simulink model "extra_tip_sim"  (Simulink 9.0)
settings: Solver=FixedStepDiscrete  StartTime=start_time  StopTime=stop_time  FixedStep=0.020  RelTol=1e-3  EnableMultiTasking=on
InitFcn:
  | extra_tip_sim_init
values from neighbouring files (symbols this model uses):
  bucketAngle = WeighDebug_TOAbucket_angle_t27    [extra_tip_sim_init.m]
  imuX = WeighDebug_TOAeef_imu_accelX_t27    [extra_tip_sim_init.m]    (also in imu_pitch_cal_sim_init.m = WeighDebug_TOAeef_imu_accelX_t194)
  imuY = WeighDebug_TOAeef_imu_accelY_t27    [extra_tip_sim_init.m]    (also in imu_pitch_cal_sim_init.m = WeighDebug_TOAeef_imu_accelY_t194)
  imuZ = WeighDebug_TOAeef_imu_accelZ_t27    [extra_tip_sim_init.m]    (also in imu_pitch_cal_sim_init.m = WeighDebug_TOAeef_imu_accelZ_t194)
  liftAngle = WeighDebug_TOAlift_angle_t27    [extra_tip_sim_init.m]    (also in imu_pitch_cal_sim_init.m = WeighDebug_TOAlift_angle_t194)
  liftCmd = WeighDebug_TOAlift_valve_cmd_t27    [extra_tip_sim_init.m]
  liftCylLength = WeighDebug_LiftCylNormLen_t27    [extra_tip_sim_init.m]    (also in imu_pitch_cal_sim_init.m = WeighDebug_LiftCylLenghtNorm_Val_t194)
  liftCylPress = WeighDebug_LiftCylPres_t27    [extra_tip_sim_init.m]    (also in imu_pitch_cal_sim_init.m = WeighDebug_LiftCylPres_t194)
  payloadTarget = TOAtestPts_toa_payload_target_final_t27    [extra_tip_sim_init.m]
  steerAng = WeighDebug_TOAsteering_angle_t27    [extra_tip_sim_init.m]    (also in imu_pitch_cal_sim_init.m = WeighDebug_TOAsteering_angle_t194)
  tiltCmd = WeighDebug_TOAtilt_valve_cmd_t27    [extra_tip_sim_init.m]
  tiltExt = WeighDebug_TOAtilt_extension_t27    [extra_tip_sim_init.m]    (also in imu_pitch_cal_sim_init.m = WeighDebug_TOAtilt_extension_t194)
  tiltHePress = WeighDebug_TOAtilt_he_pressure_t27    [extra_tip_sim_init.m]    (also in imu_pitch_cal_sim_init.m = WeighDebug_TOAtilt_he_pressure_t194)
  tiltRePress = WeighDebug_TOAtilt_re_pressure_t27    [extra_tip_sim_init.m]    (also in imu_pitch_cal_sim_init.m = WeighDebug_TOAtilt_re_pressure_t194)
  time = t27    [extra_tip_sim_init.m]    (also in imu_pitch_cal_sim_init.m = t194)
  time2 = t27    [extra_tip_sim_init.m]    (also in imu_pitch_cal_sim_init.m = t194)
  time3 = t28    [extra_tip_sim_init.m]
  toolMass = WeighDebug_TOAtool_mass_t28    [extra_tip_sim_init.m]
  unlatchTrigger = WeighDebug_TOAunlatch_trigger_t27    [extra_tip_sim_init.m]
undefined symbols (not defined in the file or in its folder): g, timestep, TipAssistLiveWeighStatus_t, TipAssistPfwStatus_t, toa_appNumber, toa_imu_lpf_cutoff_hz, toa_imuBasicOrient, toa_liftBoreDia, toa_liveLpfCutoffHz, toa_pfwLpfCutoffHz, toa_ratedPayload, toa_tiltBoreDia, toa_tiltNumCyl, toa_tiltRodDia, toa_toolBcLength
libraries: simulink x28, lib_CATutils_Utilities_ApplyName_v2 x15, lib_CATutils_Filters_1Pole_LowPass x3, tip_assist_lib x3, lib_CATutils_Timer_Countdown x3, simulink_extras x2, lib_CATutils_Override x1
(part 2 of 3)

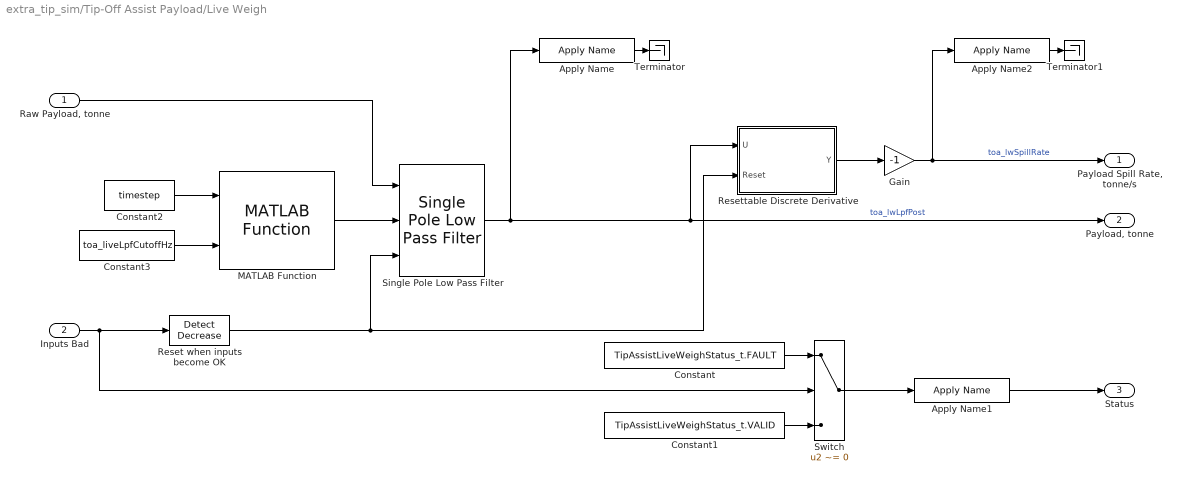
== system extra_tip_sim/Tip-Off Assist Payload/Live Weigh ==
  "Raw Payload, tonne" : Inport
  Inputs Bad : Inport  Port=2
  Apply Name : lib_CATutils_Utilities_ApplyName_v2/Apply Name  sigLabel='toa_lwLpfPost2'  enTst=true
  Apply Name1 : lib_CATutils_Utilities_ApplyName_v2/Apply Name  sigLabel='toa_lwStatus'  enTst=true
  Apply Name2 : lib_CATutils_Utilities_ApplyName_v2/Apply Name  sigLabel='toa_lwSpillRate2'  enTst=true
  Constant : Constant  Value=TipAssistLiveWeighStatus_t.FAULT  SampleTime=-1
  Constant1 : Constant  Value=TipAssistLiveWeighStatus_t.VALID  SampleTime=-1
  Constant2 : Constant  Value=timestep  SampleTime=timestep
  Constant3 : Constant  Value=toa_liveLpfCutoffHz  SampleTime=timestep
  Gain : Gain  Gain=-1
  MATLAB Function : tip_assist_lib/MATLAB Function
      settings: SourceProductName=Stateflow  SourceProductBaseCode=SF
  Reset when inputs become OK : simulink/Logic and Bit Operations/Detect Decrease  vinit=0  OutDataTypeStr=boolean
  Resettable Discrete Derivative : Subsystem  mask(Discrete Derivative){gainval=1, InputProcessing=Inherited, OutMin=[], OutMax=[], OutDataTypeStr=single, OutputDataTypeScalingMode=single, OutDataType=fixdt(1, 16), OutScaling=2^-10, LockScale=off, RndMeth=Floor, DoSatur=off}
      mask prompts: gainval "Simulink:masks:GainValue_MP"; InputProcessing "Simulink:masks:InputProcessing_MP"; OutMin "Simulink:masks:OutputMinimum_MP"; OutMax "Simulink:masks:OutputMaximum_MP"; OutDataTypeStr "Simulink:masks:OutputDataType_MP"; OutputDataTypeScalingMode "Simulink:masks:OutputDataTypeMode_MP"; OutDataType "Simulink:masks:OutputDataTypeegFixdt116Fixdtsingle_MP"; OutScaling "Simulink:masks:OutputScalingSlopeEg29OrSlopeBias_MP"; LockScale "Simulink:masks:LockOutputDataTypeAgainstFxpTools_MP"; RndMeth "Simulink:masks:IntegerRoundingMode_MP"; DoSatur "Simulink:masks:SaturateToMaxOrMinWhenOverflowsOccur_MP"
      mask help: Simulink:masks:DiscreteDerivative_MD
      mask init:
      | blkH = gcbh;
      | blkName = getfullname(blkH);
      | 
      | if (gainval == 0.0)
      |     %avoid divide by zero warning
      |     inverseGainval = inf;
      | else
      |     inverseGainval = 1.0/double(gainval);
      | end
      | 
      | if isequal(OutDataTypeStr, 'Inherit: Inherit via internal rule')
      |     diffDT   = 'Inherit: Inherit via back propagation';
      |     tsampDT  = 'Inherit: Inherit via internal rule';
      |     tsampImp = 'Offline Scaling Adjustment';
      | else    
      |     diffDT   = OutDataTypeStr;
      |     tsampDT  = 'Inherit: Inherit via back propagation';
      |     tsampImp = 'Online Calculations';
      | end
      | 
      | if ~strcmp(get_param(bdroot(blkH),'SimulationStatus'), 'running')
      |     set_param([blkName,'/Diff'], ...
      |               'RndMeth',RndMeth, ...
      | 	          'DoSatur',DoSatur);
      |     set_param([blkName,'/TSamp'], ...
      |               'OutDataTypeStr',tsampDT, ...
      |               'RndMeth',RndMeth, ...
      |               'DoSatur',DoSatur, ...
      |               'TsampMathImp',tsampImp);
      | end
      | 
      | set_param([blkName,'/Resettable Delay'], ...
      | 	'InputProcessing',InputProcessing);
      mask TypeOptions InputProcessing: Simulink:masks:ColumnsAsChannelsFrameBased | Simulink:masks:ElementsAsChannelsSampleBased | Simulink:masks:Inherited
      mask Callback OutDataTypeStr: fixptdialog(gcbh)
      mask TypeOptions OutputDataTypeScalingMode: double | single | int8 | uint8 | int16 | uint16 | int32 | uint32 | Specify via dialog | Inherit via internal rule | Inherit via back propagation
      mask Callback OutputDataTypeScalingMode: fixptdialog(gcbh)
      mask Callback OutDataType: fixptdialog(gcbh)
      mask TypeOptions RndMeth: Simulink:masks:Ceiling | Simulink:masks:Convergent | Simulink:masks:Floor | Simulink:masks:Nearest | Simulink:masks:Round | Simulink:masks:Simplest | Simulink:masks:Zero
      mask Display: text(0.5, 0.5, 'K (z-1)', 'horizontalAlignment', 'center', 'verticalAlignment', 'bottom');text(0.5, 0.5, 'Ts z', 'horizontalAlignment', 'center', 'verticalAlignment', 'top');plot([0.3 0.7],[0.5 0.5]);
  Single Pole Low Pass Filter : lib_CATutils_Filters_1Pole_LowPass/Single Pole Low Pass Filter  extFactor=on  extReset=on  incIntWordSize=off  mainInternalRes=off  filtFactor=.0001
  Switch : Switch  Criteria=u2 ~= 0
  Terminator : Terminator
  Terminator1 : Terminator
  "Payload Spill Rate, tonne/s" : Outport
  "Payload, tonne" : Outport  Port=2
  Status : Outport  Port=3
  wires:
  Apply Name2/1 -> Terminator1/1
  Apply Name/1 -> Terminator/1
  Gain/1 -> Apply Name2/1, "Payload Spill Rate, tonne/s"/1  "toa_lwSpillRate"
  Resettable Discrete Derivative/1(Y) -> Gain/1
  Apply Name1/1 -> Status/1
  Constant3/1 -> MATLAB Function/2
  Constant2/1 -> MATLAB Function/1
  Switch/1 -> Apply Name1/1
  Constant1/1 -> Switch/3
  Constant/1 -> Switch/1
  "Raw Payload, tonne"/1 -> Single Pole Low Pass Filter/1
  Inputs Bad/1 -> Reset when inputs become OK/1, Switch/2
  Reset when inputs become OK/1 -> Single Pole Low Pass Filter/3, Resettable Discrete Derivative/2(Reset)
  MATLAB Function/1 -> Single Pole Low Pass Filter/2
  Single Pole Low Pass Filter/1 -> "Payload, tonne"/1, Resettable Discrete Derivative/1(U), Apply Name/1  "toa_lwLpfPost"

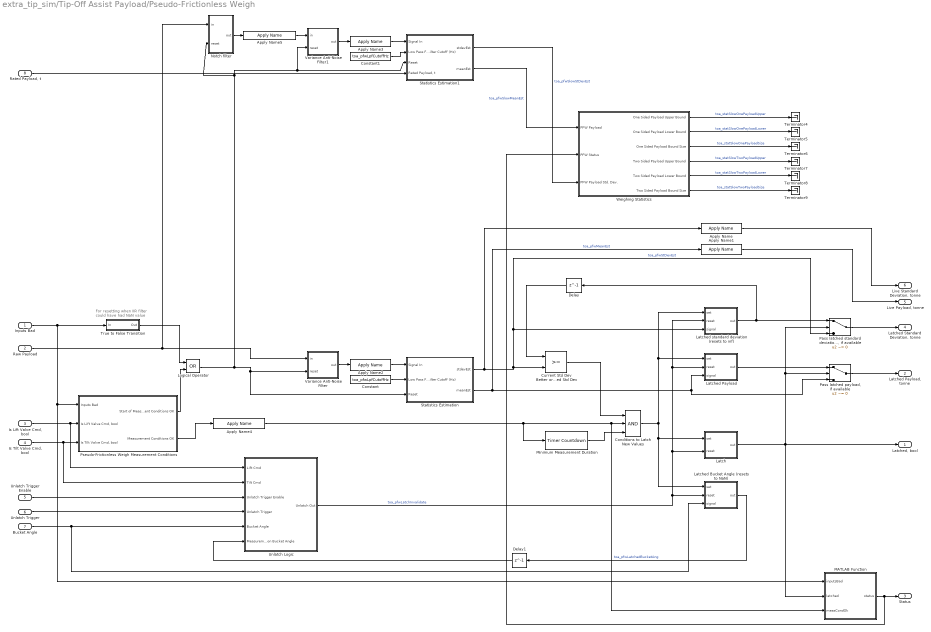
== system extra_tip_sim/Tip-Off Assist Payload/Pseudo-Frictionless Weigh ==
  note: For resetting when IIR filter could have had NaN value
  Inputs Bad : Inport
  Raw Payload : Inport  Port=2
  "Is Lift Valve Cmd, bool" : Inport  Port=3
  "Is Tilt Valve Cmd, bool" : Inport  Port=4
  Unlatch Trigger Enable : Inport  Port=5
  Unlatch Trigger : Inport  Port=6
  Bucket Angle : Inport  Port=7
  "Rated Payload, t" : Inport  Port=8
  Apply Name : lib_CATutils_Utilities_ApplyName_v2/Apply Name  sigLabel='toa_pfwLiveStDev'  enTst=true
  Apply Name1 : lib_CATutils_Utilities_ApplyName_v2/Apply Name  sigLabel='toa_pfwLiveMean'  enTst=true
  Apply Name2 : lib_CATutils_Utilities_ApplyName_v2/Apply Name  sigLabel='toa_pfwPayloadFilt'  enTst=true
  Apply Name3 : lib_CATutils_Utilities_ApplyName_v2/Apply Name  sigLabel='toa_pfwPayloadFilt'  enTst=true
  Apply Name4 : lib_CATutils_Utilities_ApplyName_v2/Apply Name  sigLabel='toa_pfwConditionsOk'  enTst=true
  Apply Name5 : lib_CATutils_Utilities_ApplyName_v2/Apply Name  sigLabel='toa_pfwPayloadNotchPost'  enTst=true
  Conditions to Latch New Values : Logic  Inputs=3
  Constant : Constant  Value=toa_pfwLpfCutoffHz
  Constant1 : Constant  Value=toa_pfwLpfCutoffHz
  Current Std Dev Better or Equal to Previously Latched Std Dev : RelationalOperator  RndMeth=Nearest  InputSameDT=on
  Delay : Delay  DelayLength=1
  Delay1 : Delay  DelayLength=1
  Latch : Subsystem  mask{mskInitialOut=0}
      mask prompts: mskInitialOut "Initial Output"
  Latched Bucket Angle (resets to NaN) : Subsystem  mask{mskInitialOut=single(nan)}
      mask prompts: mskInitialOut "Initial Output and Reset Value"
  Latched Payload : Subsystem  mask{mskInitialOut=nan}
      mask prompts: mskInitialOut "Initial Output and Reset Value"
  Latched standard deviation (resets to inf) : Subsystem  mask{mskInitialOut=single(inf)}
      mask prompts: mskInitialOut "Initial Output and Reset Value"
  Logical Operator : Logic  Operator=OR  AllPortsSameDT=off  OutDataTypeStr=boolean
  MATLAB Function : MATLAB Function  TreatAsAtomicUnit=on
  Minimum Measurement Duration : lib_CATutils_Timer_Countdown/Timer Countdown  initTime=toa_pfw_min_meas_duration  maxTime=400  timingInput=True  expiredOutput=True  initState=False
  Notch filter : Subsystem
  "Pass latched payload, if available" : Switch  Criteria=u2 ~= 0
  "Pass latched standard deviation, if available" : Switch  Criteria=u2 ~= 0
  Pseudo-Frictionless Weigh Measurement Conditions : Subsystem
  Statistics Estimation : Subsystem
  Statistics Estimation1 : Subsystem
  Terminator{4..9} (6 alike) : Terminator
  True to False Transition : Subsystem
  Unlatch Logic : Subsystem
  Variance Anti-Noise Filter : Subsystem
  Variance Anti-Noise Filter1 : Subsystem
  Weighing Statistics : Subsystem
  "Latched, bool" : Outport
  "Latched Payload, tonne" : Outport  Port=2
  Status : Outport  Port=3
  "Latched Standard Deviation, tonne" : Outport  Port=4
  "Live Payload, tonne" : Outport  Port=5
  "Live Standard Deviation, tonne" : Outport  Port=6
  wires:
  Apply Name1/1 -> "Live Payload, tonne"/1
  Apply Name/1 -> "Live Standard Deviation, tonne"/1
  Unlatch Trigger Enable/1 -> Unlatch Logic/3(Unlatch Trigger Enable)
  Delay1/1 -> Unlatch Logic/6(Measurement Condition Bucket Angle)
  Unlatch Trigger/1 -> Unlatch Logic/4(Unlatch Trigger)
  Latched Bucket Angle (resets to NaN)/1(out) -> Delay1/1  "toa_pfwLatchedBucketAng"
  Bucket Angle/1 -> Unlatch Logic/5(Bucket Angle), Latched Bucket Angle (resets to NaN)/3(signal)
  Logical Operator/1 -> Notch filter/2(reset), Variance Anti-Noise Filter1/2(reset), Statistics Estimation1/3(Reset), Statistics Estimation/3(Reset), Variance Anti-Noise Filter/2(reset)
  True to False Transition/1(Out) -> Logical Operator/1
  Constant/1 -> Statistics Estimation/2(Low Pass Filter Cutoff (Hz))
  Inputs Bad/1 -> True to False Transition/1(In), Pseudo-Frictionless Weigh Measurement Conditions/1(Inputs Bad), MATLAB Function/1(inputsBad)
  "Is Lift Valve Cmd, bool"/1 -> Pseudo-Frictionless Weigh Measurement Conditions/2("Is Lift Valve Cmd, bool"), Unlatch Logic/1(Lift Cmd)
  Conditions to Latch New Values/1 -> Latched standard deviation (resets to inf)/1(set), Latched Payload/1(set), Latch/1(set), Latched Bucket Angle (resets to NaN)/1(set)
  Latch/1(out) -> MATLAB Function/2(latched), "Latched, bool"/1, "Pass latched payload, if available"/2, "Pass latched standard deviation, if available"/2
  Latched Payload/1(out) -> "Pass latched payload, if available"/1
  Latched standard deviation (resets to inf)/1(out) -> "Pass latched standard deviation, if available"/1, Delay/1
  Minimum Measurement Duration/1 -> Conditions to Latch New Values/3
  Current Std Dev Better or Equal to Previously Latched Std Dev/1 -> Conditions to Latch New Values/1
  Delay/1 -> Current Std Dev Better or Equal to Previously Latched Std Dev/1
  Pseudo-Frictionless Weigh Measurement Conditions/2(Measurement Conditions OK) -> Apply Name4/1
  Pseudo-Frictionless Weigh Measurement Conditions/1(Start of Measurement Conditions OK) -> Logical Operator/2
  "Is Tilt Valve Cmd, bool"/1 -> Pseudo-Frictionless Weigh Measurement Conditions/3("Is Tilt Valve Cmd, bool"), Unlatch Logic/2(Tilt Cmd)
  Variance Anti-Noise Filter/1(out) -> Apply Name2/1
  "Pass latched payload, if available"/1 -> "Latched Payload, tonne"/1
  "Pass latched standard deviation, if available"/1 -> "Latched Standard Deviation, tonne"/1
  MATLAB Function/1(status) -> Weighing Statistics/2(PFW Status), Status/1
  Statistics Estimation/1(stdevEst) -> Current Std Dev Better or Equal to Previously Latched Std Dev/2, Latched standard deviation (resets to inf)/3(signal), "Pass latched standard deviation, if available"/3, Apply Name/1  "toa_pfwStDevEst"
  Statistics Estimation/2(meanEst) -> "Pass latched payload, if available"/3, Latched Payload/3(signal), Apply Name1/1  "toa_pfwMeanEst"
  Apply Name2/1 -> Statistics Estimation/1(Signal In)
  Raw Payload/1 -> Notch filter/1(in), Variance Anti-Noise Filter/1(in)
  Apply Name4/1 -> Minimum Measurement Duration/1, MATLAB Function/3(measCondOk), Conditions to Latch New Values/2
  Unlatch Logic/1(Unlatch Out) -> Latched Bucket Angle (resets to NaN)/2(reset), Latch/2(reset), Latched Payload/2(reset), Latched standard deviation (resets to inf)/2(reset)  "toa_pfwLatchInvalidate"
  Apply Name5/1 -> Variance Anti-Noise Filter1/1(in)
  Notch filter/1(out) -> Apply Name5/1
  Variance Anti-Noise Filter1/1(out) -> Apply Name3/1
  Constant1/1 -> Statistics Estimation1/2(Low Pass Filter Cutoff (Hz))
  Apply Name3/1 -> Statistics Estimation1/1(Signal In)
  Statistics Estimation1/1(stdevEst) -> Weighing Statistics/3(PFW Payload Std. Dev.)  "toa_pfwSlowStDevEst"
  Statistics Estimation1/2(meanEst) -> Weighing Statistics/1(PFW Payload)  "toa_pfwSlowMeanEst"
  Weighing Statistics/5(Two Sided Payload Lower Bound) -> Terminator8/1  "toa_statSlowTwoPayloadLower"
  Weighing Statistics/4(Two Sided Payload Upper Bound) -> Terminator7/1  "toa_statSlowTwoPayloadUpper"
  Weighing Statistics/6(Two Sided Payload Bound Size) -> Terminator9/1  "toa_statSlowTwoPayloadSize"
  Weighing Statistics/1(One Sided Payload Upper Bound) -> Terminator4/1  "toa_statSlowOnePayloadUpper"
  Weighing Statistics/2(One Sided Payload Lower Bound) -> Terminator5/1  "toa_statSlowOnePayloadLower"
  Weighing Statistics/3(One Sided Payload Bound Size) -> Terminator6/1  "toa_statSlowOnePayloadSize"
  "Rated Payload, t"/1 -> Statistics Estimation1/4("Rated Payload, t")

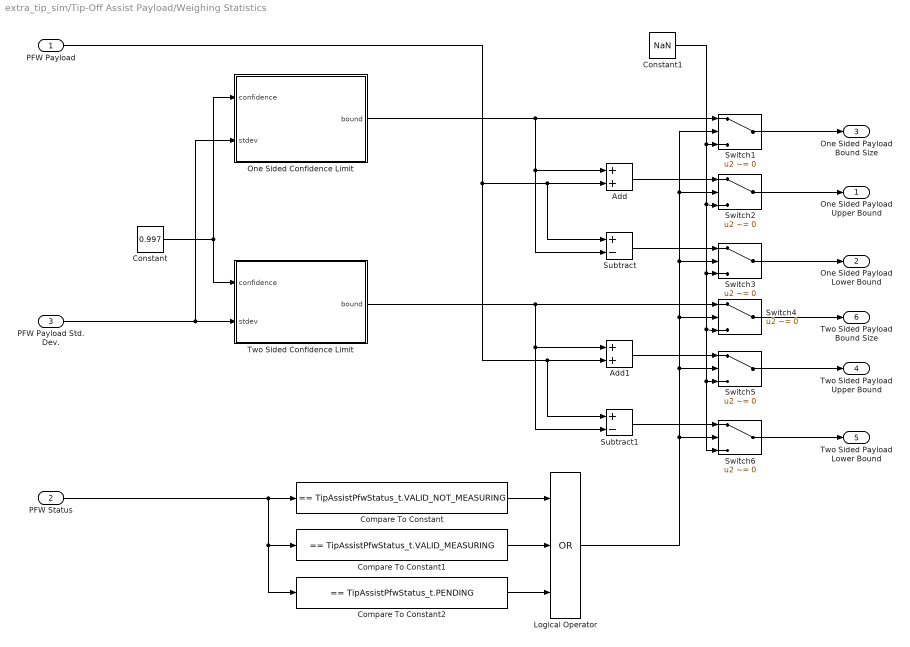
== system extra_tip_sim/Tip-Off Assist Payload/Weighing Statistics ==
  PFW Payload : Inport
  PFW Status : Inport  Port=2
  PFW Payload Std. Dev. : Inport  Port=3
  Add : Sum
  Add1 : Sum
  Compare To Constant : simulink/Logic and Bit Operations/Compare To Constant  relop===  const=TipAssistPfwStatus_t.VALID_NOT_MEASURING  OutDataTypeStr=boolean
  Compare To Constant1 : simulink/Logic and Bit Operations/Compare To Constant  relop===  const=TipAssistPfwStatus_t.VALID_MEASURING  OutDataTypeStr=boolean
  Compare To Constant2 : simulink/Logic and Bit Operations/Compare To Constant  relop===  const=TipAssistPfwStatus_t.PENDING  OutDataTypeStr=boolean
  Constant : Constant  Value=0.997
  Constant1 : Constant  Value=NaN  OutDataTypeStr=single
  Logical Operator : Logic  Operator=OR  Inputs=3  AllPortsSameDT=off  OutDataTypeStr=boolean
  One Sided Confidence Limit : MATLAB Function  TreatAsAtomicUnit=on
  Subtract : Sum  Inputs=+-
  Subtract1 : Sum  Inputs=+-
  Switch{1..6} (6 alike) : Switch  Criteria=u2 ~= 0
  Two Sided Confidence Limit : MATLAB Function  TreatAsAtomicUnit=on
  One Sided Payload Upper Bound : Outport
  One Sided Payload Lower Bound : Outport  Port=2
  One Sided Payload Bound Size : Outport  Port=3
  Two Sided Payload Upper Bound : Outport  Port=4
  Two Sided Payload Lower Bound : Outport  Port=5
  Two Sided Payload Bound Size : Outport  Port=6
  wires:
  Compare To Constant2/1 -> Logical Operator/3
  Compare To Constant1/1 -> Logical Operator/2
  Compare To Constant/1 -> Logical Operator/1
  Logical Operator/1 -> Switch1/2, Switch2/2, Switch3/2, Switch4/2, Switch5/2, Switch6/2
  Switch6/1 -> Two Sided Payload Lower Bound/1
  Switch5/1 -> Two Sided Payload Upper Bound/1
  Switch4/1 -> Two Sided Payload Bound Size/1
  Switch3/1 -> One Sided Payload Lower Bound/1
  Switch2/1 -> One Sided Payload Upper Bound/1
  Switch1/1 -> One Sided Payload Bound Size/1
  Constant1/1 -> Switch6/3, Switch5/3, Switch4/3, Switch3/3, Switch2/3, Switch1/3
  Constant/1 -> Two Sided Confidence Limit/1(confidence), One Sided Confidence Limit/1(confidence)
  PFW Payload Std. Dev./1 -> One Sided Confidence Limit/2(stdev), Two Sided Confidence Limit/2(stdev)
  PFW Status/1 -> Compare To Constant2/1, Compare To Constant1/1, Compare To Constant/1
  Two Sided Confidence Limit/1(bound) -> Switch4/1, Add1/1, Subtract1/2
  PFW Payload/1 -> Add/2, Subtract/1, Add1/2, Subtract1/1
  Subtract1/1 -> Switch6/1
  Add1/1 -> Switch5/1
  Subtract/1 -> Switch3/1
  One Sided Confidence Limit/1(bound) -> Switch1/1, Add/1, Subtract/2
  Add/1 -> Switch2/1

== system extra_tip_sim/EEF IMU to NEEF gravity vector/imu lpf x1/Filter Factor Calc ==
  Cutoff (Hz) : Inport
  Constant1 : Constant  Value=-2 * pi * timestep  OutDataTypeStr=single
  Constant3 : Constant  OutDataTypeStr=single
  Math Function : Math  OutputSignalType=real  SaturateOnIntegerOverflow=on
  Multiply : Product  SaturateOnIntegerOverflow=on  RndMeth=Zero  InputSameDT=on  OutDataTypeStr=Inherit: Same as first input
  Subtract : Sum  Inputs=|+-  SaturateOnIntegerOverflow=on  InputSameDT=on  OutDataTypeStr=Inherit: Same as first input
  Filter Factor : Outport
  wires:
  Constant1/1 -> Multiply/2
  Math Function/1 -> Subtract/2
  Multiply/1 -> Math Function/1
  Constant3/1 -> Subtract/1
  Subtract/1 -> Filter Factor/1
  Cutoff (Hz)/1 -> Multiply/1

== system extra_tip_sim/Tip-Off Assist Payload/Live Weigh/Resettable Discrete Derivative ==
  note: ( U(k) - U(k-1) )
  note: U(k)
  U : Inport
  Reset : Inport  Port=2
  Data Type Duplicate : DataTypeDuplicate  DisableCoverage=on  NumInputPorts=3
  Diff : Sum  Description=Add in CPU  Inputs=+-  OutMin=OutMin  OutMax=OutMax  OutDataTypeStr=diffDT
  Resettable Delay : Delay  DelayLength=1  InitialConditionSource=Input port  ExternalReset=Level hold  InputProcessing=Inherited
      settings: InputPortMap=u0,r5,p4
  TSamp : SampleTimeMath  DisableCoverage=on  TsampMathOp=/  weightValue=inverseGainval  OutDataTypeStr=Inherit: Inherit via back propagation
  Y : Outport  OutMin=OutMin  OutMax=OutMax  InitialOutput=0
  wires:
  Reset/1 -> Resettable Delay/2
  U/1 -> TSamp/1
  Resettable Delay/1 -> Diff/2, Data Type Duplicate/3  "U(k-1)"
  Diff/1 -> Y/1, Data Type Duplicate/1
  TSamp/1 -> Diff/1, Data Type Duplicate/2, Resettable Delay/3, Resettable Delay/1

== system extra_tip_sim/Tip-Off Assist Payload/Pseudo-Frictionless Weigh/Latch ==
  set : Inport
  reset : Inport  Port=2
  Unit Delay : UnitDelay  InitialCondition=mskInitialOut  SampleTime=-1
      settings: AttributesFormatString=IC: %<X0>
  false : Constant  Value=0  OutDataTypeStr=boolean
  resetSwitch : Switch  Criteria=u2 ~= 0  InputSameDT=on
      settings: AttributesFormatString=%<Criteria>
  setSwitch : Switch  Criteria=u2 ~= 0  InputSameDT=on
      settings: AttributesFormatString=%<Criteria>
  true : Constant  OutDataTypeStr=boolean
  out : Outport
  wires:
  reset/1 -> resetSwitch/2
  setSwitch/1 -> resetSwitch/3
  set/1 -> setSwitch/2
  false/1 -> resetSwitch/1
  true/1 -> setSwitch/1
  resetSwitch/1 -> out/1, Unit Delay/1
  Unit Delay/1 -> setSwitch/3

== system extra_tip_sim/Tip-Off Assist Payload/Pseudo-Frictionless Weigh/Latched Bucket Angle (resets to NaN) ==
  set : Inport
  reset : Inport  Port=2
  signal : Inport  Port=3
  Unit Delay : UnitDelay  InitialCondition=mskInitialOut  SampleTime=-1
      settings: AttributesFormatString=IC: %<X0>
  false : Constant  Value=mskInitialOut  OutDataTypeStr=Inherit: Inherit via back propagation  SampleTime=-1
  resetSwitch : Switch  Criteria=u2 ~= 0  InputSameDT=on
      settings: AttributesFormatString=%<Criteria>
  setSwitch : Switch  Criteria=u2 ~= 0  InputSameDT=on
      settings: AttributesFormatString=%<Criteria>
  out : Outport
  wires:
  reset/1 -> resetSwitch/2
  setSwitch/1 -> resetSwitch/3
  set/1 -> setSwitch/2
  false/1 -> resetSwitch/1
  signal/1 -> setSwitch/1
  resetSwitch/1 -> out/1, Unit Delay/1
  Unit Delay/1 -> setSwitch/3

== system extra_tip_sim/Tip-Off Assist Payload/Pseudo-Frictionless Weigh/Latched Payload ==
  set : Inport
  reset : Inport  Port=2
  signal : Inport  Port=3
  Unit Delay : UnitDelay  InitialCondition=mskInitialOut  SampleTime=-1
      settings: AttributesFormatString=IC: %<X0>
  false : Constant  Value=mskInitialOut  OutDataTypeStr=Inherit: Inherit via back propagation  SampleTime=-1
  resetSwitch : Switch  Criteria=u2 ~= 0  InputSameDT=on
      settings: AttributesFormatString=%<Criteria>
  setSwitch : Switch  Criteria=u2 ~= 0  InputSameDT=on
      settings: AttributesFormatString=%<Criteria>
  out : Outport
  wires:
  Unit Delay/1 -> setSwitch/3
  resetSwitch/1 -> Unit Delay/1, out/1
  signal/1 -> setSwitch/1
  false/1 -> resetSwitch/1
  set/1 -> setSwitch/2
  setSwitch/1 -> resetSwitch/3
  reset/1 -> resetSwitch/2

== system extra_tip_sim/Tip-Off Assist Payload/Pseudo-Frictionless Weigh/Latched standard deviation (resets to inf) ==
  set : Inport
  reset : Inport  Port=2
  signal : Inport  Port=3
  Unit Delay : UnitDelay  InitialCondition=mskInitialOut  SampleTime=-1
      settings: AttributesFormatString=IC: %<X0>
  false : Constant  Value=mskInitialOut  OutDataTypeStr=Inherit: Inherit via back propagation  SampleTime=-1
  resetSwitch : Switch  Criteria=u2 ~= 0  InputSameDT=on
      settings: AttributesFormatString=%<Criteria>
  setSwitch : Switch  Criteria=u2 ~= 0  InputSameDT=on
      settings: AttributesFormatString=%<Criteria>
  out : Outport
  wires:
  reset/1 -> resetSwitch/2
  setSwitch/1 -> resetSwitch/3
  set/1 -> setSwitch/2
  false/1 -> resetSwitch/1
  signal/1 -> setSwitch/1
  resetSwitch/1 -> out/1, Unit Delay/1
  Unit Delay/1 -> setSwitch/3

== system extra_tip_sim/Tip-Off Assist Payload/Pseudo-Frictionless Weigh/Notch filter ==
  in : Inport
  reset : Inport  Port=2
  NotchFilter : Subsystem  mask{mskCutoffFreqRadPerSec=5.0}
      mask prompts: mskCutoffFreqRadPerSec "Cutoff Frequency (rad/s)"
      settings: AttributesFormatString=cf: %<mskCutoffFreqRadPerSec>
  NotchFilter1 : Subsystem  mask{mskCutoffFreqRadPerSec=7.5}
      mask prompts: mskCutoffFreqRadPerSec "Cutoff Frequency (rad/s)"
      settings: AttributesFormatString=cf: %<mskCutoffFreqRadPerSec>
  NotchFilter2 : Subsystem  mask{mskCutoffFreqRadPerSec=12.0}
      mask prompts: mskCutoffFreqRadPerSec "Cutoff Frequency (rad/s)"
      settings: AttributesFormatString=cf: %<mskCutoffFreqRadPerSec>
  out : Outport
  wires:
  NotchFilter/1(filtered) -> NotchFilter1/1(raw)
  NotchFilter1/1(filtered) -> NotchFilter2/1(raw)
  reset/1 -> NotchFilter2/2(reset), NotchFilter1/2(reset), NotchFilter/2(reset)
  in/1 -> NotchFilter/1(raw)
  NotchFilter2/1(filtered) -> out/1

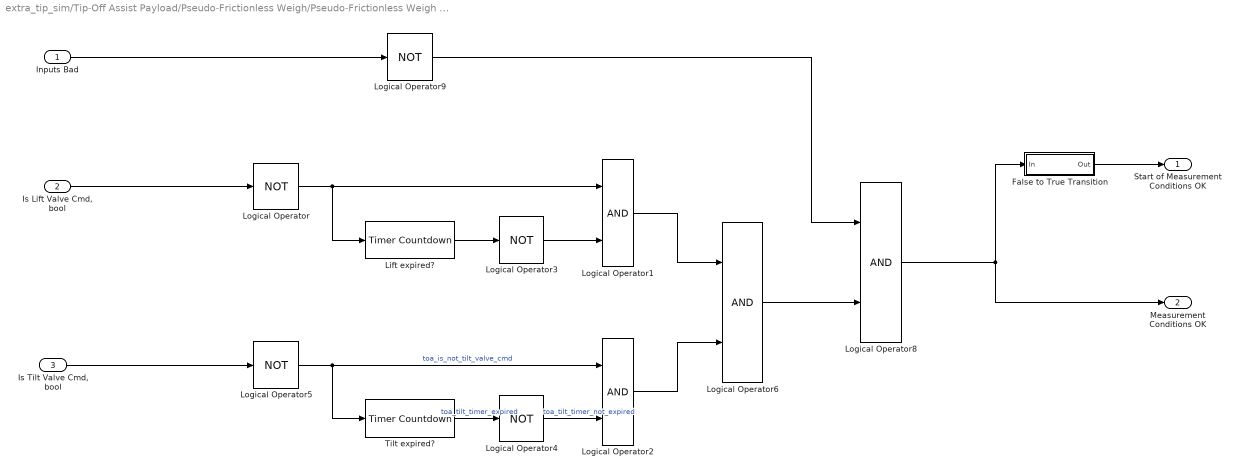
== system extra_tip_sim/Tip-Off Assist Payload/Pseudo-Frictionless Weigh/Pseudo-Frictionless Weigh Measurement Conditions ==
  Inputs Bad : Inport
  "Is Lift Valve Cmd, bool" : Inport  Port=2
  "Is Tilt Valve Cmd, bool" : Inport  Port=3
  False to True Transition : Subsystem
  Lift expired? : lib_CATutils_Timer_Countdown/Timer Countdown  initTime=toa_pfw_time_limit  maxTime=400  timingInput=True  expiredOutput=True  initState=False
  Logical Operator{,3..5,9} (5 alike) : Logic  Operator=NOT
  Logical Operator{1..2,6,8} (4 alike) : Logic
  Tilt expired? : lib_CATutils_Timer_Countdown/Timer Countdown  initTime=toa_pfw_time_limit  maxTime=400  timingInput=True  expiredOutput=True  initState=False
  Start of Measurement Conditions OK : Outport
  Measurement Conditions OK : Outport  Port=2
  wires:
  Logical Operator9/1 -> Logical Operator8/1
  Inputs Bad/1 -> Logical Operator9/1
  Logical Operator6/1 -> Logical Operator8/2
  "Is Tilt Valve Cmd, bool"/1 -> Logical Operator5/1
  "Is Lift Valve Cmd, bool"/1 -> Logical Operator/1
  Logical Operator/1 -> Lift expired?/1, Logical Operator1/1
  Tilt expired?/1 -> Logical Operator4/1  "toa_tilt_timer_expired"
  Logical Operator5/1 -> Logical Operator2/1, Tilt expired?/1  "toa_is_not_tilt_valve_cmd"
  Lift expired?/1 -> Logical Operator3/1
  Logical Operator3/1 -> Logical Operator1/2
  Logical Operator4/1 -> Logical Operator2/2  "toa_tilt_timer_not_expired"
  Logical Operator1/1 -> Logical Operator6/1
  Logical Operator2/1 -> Logical Operator6/2
  Logical Operator8/1 -> False to True Transition/1(In), Measurement Conditions OK/1
  False to True Transition/1(Out) -> Start of Measurement Conditions OK/1

== system extra_tip_sim/Tip-Off Assist Payload/Pseudo-Frictionless Weigh/Statistics Estimation ==
  Signal In : Inport
  Low Pass Filter Cutoff (Hz) : Inport  Port=2
  Reset : Inport  Port=3
  Constant2 : Constant  Value=timestep  SampleTime=timestep
  MATLAB Function : MATLAB Function  TreatAsAtomicUnit=on
  MATLAB Function1 : tip_assist_lib/MATLAB Function
  stdevEst : Outport
  meanEst : Outport  Port=2
  wires:
  Reset/1 -> MATLAB Function/3(reset)
  MATLAB Function1/1 -> MATLAB Function/2(filterFactor)
  Low Pass Filter Cutoff (Hz)/1 -> MATLAB Function1/2
  Constant2/1 -> MATLAB Function1/1
  MATLAB Function/2(stdevEst) -> stdevEst/1
  MATLAB Function/1(meanEst) -> meanEst/1
  Signal In/1 -> MATLAB Function/1(newSample)

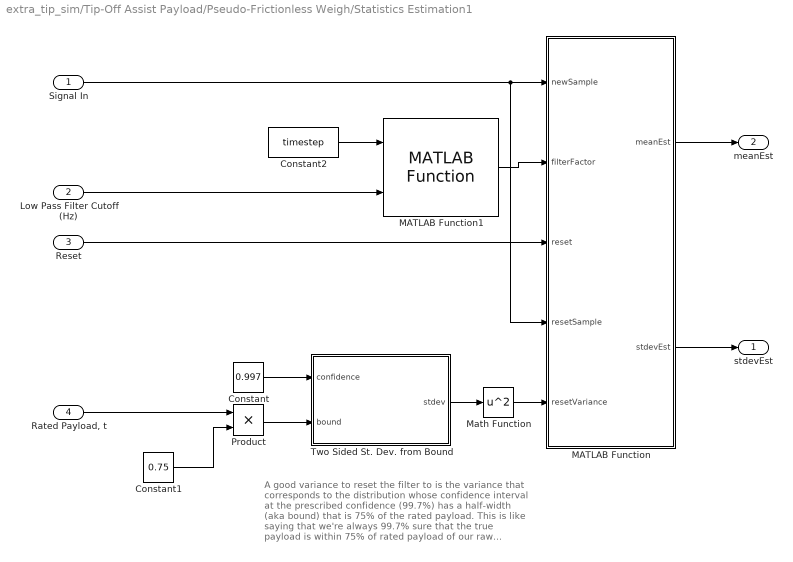
== system extra_tip_sim/Tip-Off Assist Payload/Pseudo-Frictionless Weigh/Statistics Estimation1 ==
  note: A good variance to reset the filter to is the variance that corresponds to the distribution whose confidence interval at the prescribed confidence (99.7%) has a half-width (aka bound) that is 75% of the rated payload.
      |
      | This is like saying that we're always 99.7% sure that the true payload is within 75% of rated payload of our raw measurement.
  Signal In : Inport
  Low Pass Filter Cutoff (Hz) : Inport  Port=2
  Reset : Inport  Port=3
  "Rated Payload, t" : Inport  Port=4
  Constant : Constant  Value=0.997  OutDataTypeStr=single  SampleTime=-1
  Constant1 : Constant  Value=0.75  OutDataTypeStr=single  SampleTime=-1
  Constant2 : Constant  Value=timestep  SampleTime=timestep
  MATLAB Function : MATLAB Function  TreatAsAtomicUnit=on
  MATLAB Function1 : tip_assist_lib/MATLAB Function
  Math Function : Math  Operator=square  SaturateOnIntegerOverflow=on
  Product : Product
  Two Sided St. Dev. from Bound : MATLAB Function  TreatAsAtomicUnit=on
  stdevEst : Outport
  meanEst : Outport  Port=2
  wires:
  Reset/1 -> MATLAB Function/3(reset)
  MATLAB Function1/1 -> MATLAB Function/2(filterFactor)
  Low Pass Filter Cutoff (Hz)/1 -> MATLAB Function1/2
  Constant2/1 -> MATLAB Function1/1
  MATLAB Function/2(stdevEst) -> stdevEst/1
  MATLAB Function/1(meanEst) -> meanEst/1
  Signal In/1 -> MATLAB Function/4(resetSample), MATLAB Function/1(newSample)
  "Rated Payload, t"/1 -> Product/1
  Constant/1 -> Two Sided St. Dev. from Bound/1(confidence)
  Math Function/1 -> MATLAB Function/5(resetVariance)
  Two Sided St. Dev. from Bound/1(stdev) -> Math Function/1
  Constant1/1 -> Product/2
  Product/1 -> Two Sided St. Dev. from Bound/2(bound)

== system extra_tip_sim/Tip-Off Assist Payload/Pseudo-Frictionless Weigh/True to False Transition ==
  In : Inport
  Compare to Constant : simulink/Logic and Bit Operations/Compare To Constant  relop===  const=0  OutDataTypeStr=boolean
      settings: AttributesFormatString=Operator: %<relop>\nConst: %<const>
  Compare to Constant1 : simulink/Logic and Bit Operations/Compare To Constant  relop===  const=1  OutDataTypeStr=boolean
      settings: AttributesFormatString=Operator: %<relop>\nConst: %<const>
  Delay1 : Delay  DelayLength=1
  Logical Operator : Logic
  Out : Outport
  wires:
  Delay1/1 -> Compare to Constant1/1
  Compare to Constant1/1 -> Logical Operator/1
  In/1 -> Delay1/1, Compare to Constant/1
  Compare to Constant/1 -> Logical Operator/2
  Logical Operator/1 -> Out/1

== system extra_tip_sim/Tip-Off Assist Payload/Pseudo-Frictionless Weigh/Unlatch Logic ==
  Lift Cmd : Inport
  Tilt Cmd : Inport  Port=2
  Unlatch Trigger Enable : Inport  Port=3
  Unlatch Trigger : Inport  Port=4
  Bucket Angle : Inport  Port=5
  Measurement Condition Bucket Angle : Inport  Port=6
  Logical Operator1 : Logic  Operator=OR  AllPortsSameDT=off  OutDataTypeStr=boolean
  Logical Operator2 : Logic  Operator=OR  AllPortsSameDT=off  OutDataTypeStr=boolean
  Not sure payload has been retained : RelationalOperator  Operator=<  RndMeth=Nearest  InputSameDT=on
  Subtract : Sum  Inputs=+-
  Switch : Switch  Criteria=u2 ~= 0
  Tolerance (deg) : Constant  OutDataTypeStr=single  SampleTime=-1
  Unlatch Out : Outport
  wires:
  Logical Operator2/1 -> Switch/3
  Tilt Cmd/1 -> Logical Operator2/2
  Lift Cmd/1 -> Logical Operator2/1
  Switch/1 -> Logical Operator1/1
  Unlatch Trigger Enable/1 -> Switch/2
  Bucket Angle/1 -> Not sure payload has been retained/1
  Subtract/1 -> Not sure payload has been retained/2
  Unlatch Trigger/1 -> Switch/1
  Tolerance (deg)/1 -> Subtract/2
  Not sure payload has been retained/1 -> Logical Operator1/2
  Logical Operator1/1 -> Unlatch Out/1
  Measurement Condition Bucket Angle/1 -> Subtract/1

== system extra_tip_sim/Tip-Off Assist Payload/Pseudo-Frictionless Weigh/Variance Anti-Noise Filter ==
  note: Per Aaron Shatters:
      | This filter was added to PCS (the CPM predecessor) because pump piston pass frequency was aliasing into the signal.  Being kind of like a discrete derivative, the variance calculation is sensitive to high frequency noise.  So this filter was added to prevent the high frequency instances of this noise.  Being a two sample moving average, it is the fastest filter that eliminated the noise.  It was not thoroughly technically examined, but it worked.  It's not clear the extent to which this is necessary here, since Pseudo-Frictionless Weigh works only when the tilt and lift valve command is zero, so the pump should not be hydraulically connected to the cylinder at this time.  The pump is also likely to be at a low stroke, so piston pass ripple amplitude should be low.
  in : Inport
  reset : Inport  Port=2
  MATLAB Function : MATLAB Function  TreatAsAtomicUnit=on
  out : Outport
  wires:
  reset/1 -> MATLAB Function/2(reset)
  in/1 -> MATLAB Function/1(u)
  MATLAB Function/1(y) -> out/1

== system extra_tip_sim/Tip-Off Assist Payload/Pseudo-Frictionless Weigh/Variance Anti-Noise Filter1 ==
  note: Per Aaron Shatters:
      | This filter was added to PCS (the CPM predecessor) because pump piston pass frequency was aliasing into the signal.  Being kind of like a discrete derivative, the variance calculation is sensitive to high frequency noise.  So this filter was added to prevent the high frequency instances of this noise.  Being a two sample moving average, it is the fastest filter that eliminated the noise.  It was not thoroughly technically examined, but it worked.  It's not clear the extent to which this is necessary here, since Pseudo-Frictionless Weigh works only when the tilt and lift valve command is zero, so the pump should not be hydraulically connected to the cylinder at this time.  The pump is also likely to be at a low stroke, so piston pass ripple amplitude should be low.
  in : Inport
  reset : Inport  Port=2
  MATLAB Function : MATLAB Function  TreatAsAtomicUnit=on
  out : Outport
  wires:
  reset/1 -> MATLAB Function/2(reset)
  in/1 -> MATLAB Function/1(u)
  MATLAB Function/1(y) -> out/1

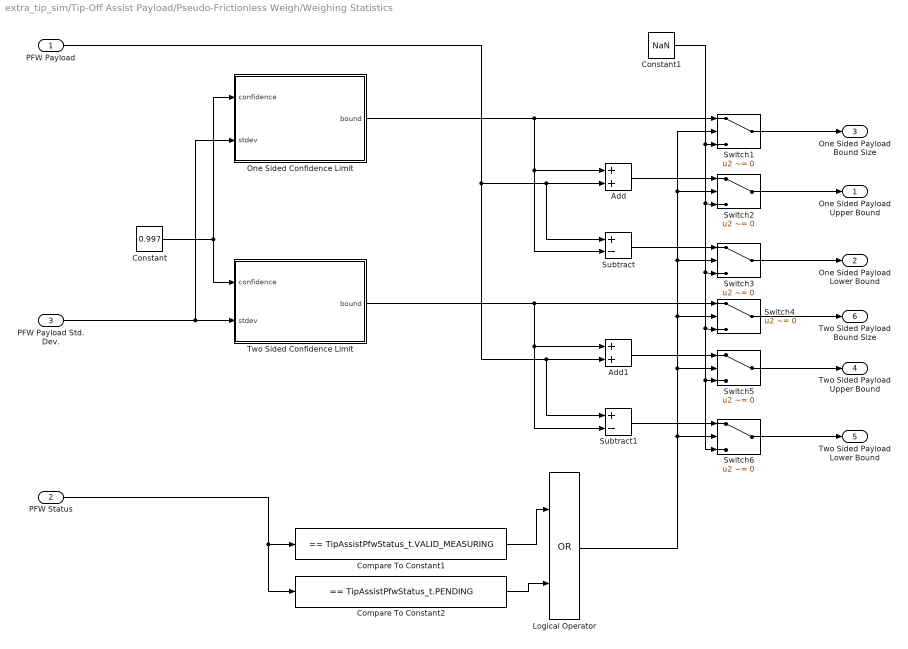
== system extra_tip_sim/Tip-Off Assist Payload/Pseudo-Frictionless Weigh/Weighing Statistics ==
  PFW Payload : Inport
  PFW Status : Inport  Port=2
  PFW Payload Std. Dev. : Inport  Port=3
  Add : Sum
  Add1 : Sum
  Compare To Constant1 : simulink/Logic and Bit Operations/Compare To Constant  relop===  const=TipAssistPfwStatus_t.VALID_MEASURING  OutDataTypeStr=boolean
  Compare To Constant2 : simulink/Logic and Bit Operations/Compare To Constant  relop===  const=TipAssistPfwStatus_t.PENDING  OutDataTypeStr=boolean
  Constant : Constant  Value=0.997
  Constant1 : Constant  Value=NaN  OutDataTypeStr=single
  Logical Operator : Logic  Operator=OR  AllPortsSameDT=off  OutDataTypeStr=boolean
  One Sided Confidence Limit : MATLAB Function  TreatAsAtomicUnit=on
  Subtract : Sum  Inputs=+-
  Subtract1 : Sum  Inputs=+-
  Switch{1..6} (6 alike) : Switch  Criteria=u2 ~= 0
  Two Sided Confidence Limit : MATLAB Function  TreatAsAtomicUnit=on
  One Sided Payload Upper Bound : Outport
  One Sided Payload Lower Bound : Outport  Port=2
  One Sided Payload Bound Size : Outport  Port=3
  Two Sided Payload Upper Bound : Outport  Port=4
  Two Sided Payload Lower Bound : Outport  Port=5
  Two Sided Payload Bound Size : Outport  Port=6
  wires:
  Compare To Constant2/1 -> Logical Operator/2
  Compare To Constant1/1 -> Logical Operator/1
  Logical Operator/1 -> Switch1/2, Switch2/2, Switch3/2, Switch4/2, Switch5/2, Switch6/2
  Switch6/1 -> Two Sided Payload Lower Bound/1
  Switch5/1 -> Two Sided Payload Upper Bound/1
  Switch4/1 -> Two Sided Payload Bound Size/1
  Switch3/1 -> One Sided Payload Lower Bound/1
  Switch2/1 -> One Sided Payload Upper Bound/1
  Switch1/1 -> One Sided Payload Bound Size/1
  Constant1/1 -> Switch6/3, Switch5/3, Switch4/3, Switch3/3, Switch2/3, Switch1/3
  Constant/1 -> Two Sided Confidence Limit/1(confidence), One Sided Confidence Limit/1(confidence)
  PFW Payload Std. Dev./1 -> One Sided Confidence Limit/2(stdev), Two Sided Confidence Limit/2(stdev)
  PFW Status/1 -> Compare To Constant2/1, Compare To Constant1/1
  Two Sided Confidence Limit/1(bound) -> Switch4/1, Add1/1, Subtract1/2
  PFW Payload/1 -> Add/2, Subtract/1, Add1/2, Subtract1/1
  Subtract1/1 -> Switch6/1
  Add1/1 -> Switch5/1
  Subtract/1 -> Switch3/1
  One Sided Confidence Limit/1(bound) -> Switch1/1, Add/1, Subtract/2
  Add/1 -> Switch2/1

== system extra_tip_sim/Tip-Off Assist Payload/Pseudo-Frictionless Weigh/Notch filter/NotchFilter ==
  raw : Inport
  reset : Inport  Port=2
  Constant : Constant  Value=mskCutoffFreqRadPerSec  OutDataTypeStr=Inherit: Inherit via back propagation
  Data Type Duplicate : DataTypeDuplicate
  Data Type Conversion : DataTypeConversion
  Data Type Conversion1 : DataTypeConversion  SaturateOnIntegerOverflow=on
  Filter : Stateflow chart  TreatAsAtomicUnit=on
  Weighted Sample Time : SampleTimeMath  TsampMathOp=Ts Only  OutDataTypeStr=Inherit: Inherit via back propagation
  filtered : Outport
  wires:
  Filter/1(filtered) -> Data Type Conversion1/1
  reset/1 -> Filter/2(reset)
  Weighted Sample Time/1 -> Filter/3(ts)
  Constant/1 -> Filter/4(cf)
  Data Type Conversion/1 -> Filter/1(raw)
  Data Type Conversion1/1 -> Data Type Duplicate/2, filtered/1
  raw/1 -> Weighted Sample Time/1, Data Type Duplicate/1, Data Type Conversion/1

== system extra_tip_sim/Tip-Off Assist Payload/Pseudo-Frictionless Weigh/Notch filter/NotchFilter1 ==
  raw : Inport
  reset : Inport  Port=2
  Constant : Constant  Value=mskCutoffFreqRadPerSec  OutDataTypeStr=Inherit: Inherit via back propagation
  Data Type Duplicate : DataTypeDuplicate
  Data Type Conversion : DataTypeConversion
  Data Type Conversion1 : DataTypeConversion  SaturateOnIntegerOverflow=on
  Filter : Stateflow chart  TreatAsAtomicUnit=on
  Weighted Sample Time : SampleTimeMath  TsampMathOp=Ts Only  OutDataTypeStr=Inherit: Inherit via back propagation
  filtered : Outport
  wires:
  Filter/1(filtered) -> Data Type Conversion1/1
  reset/1 -> Filter/2(reset)
  Weighted Sample Time/1 -> Filter/3(ts)
  Constant/1 -> Filter/4(cf)
  Data Type Conversion/1 -> Filter/1(raw)
  Data Type Conversion1/1 -> Data Type Duplicate/2, filtered/1
  raw/1 -> Weighted Sample Time/1, Data Type Duplicate/1, Data Type Conversion/1

== system extra_tip_sim/Tip-Off Assist Payload/Pseudo-Frictionless Weigh/Notch filter/NotchFilter2 ==
  raw : Inport
  reset : Inport  Port=2
  Constant : Constant  Value=mskCutoffFreqRadPerSec  OutDataTypeStr=Inherit: Inherit via back propagation
  Data Type Duplicate : DataTypeDuplicate
  Data Type Conversion : DataTypeConversion
  Data Type Conversion1 : DataTypeConversion  SaturateOnIntegerOverflow=on
  Filter : Stateflow chart  TreatAsAtomicUnit=on
  Weighted Sample Time : SampleTimeMath  TsampMathOp=Ts Only  OutDataTypeStr=Inherit: Inherit via back propagation
  filtered : Outport
  wires:
  Filter/1(filtered) -> Data Type Conversion1/1
  reset/1 -> Filter/2(reset)
  Weighted Sample Time/1 -> Filter/3(ts)
  Constant/1 -> Filter/4(cf)
  Data Type Conversion/1 -> Filter/1(raw)
  Data Type Conversion1/1 -> Data Type Duplicate/2, filtered/1
  raw/1 -> Weighted Sample Time/1, Data Type Duplicate/1, Data Type Conversion/1

== system extra_tip_sim/Tip-Off Assist Payload/Pseudo-Frictionless Weigh/Pseudo-Frictionless Weigh Measurement Conditions/False to True Transition ==
  In : Inport
  Compare to Constant : simulink/Logic and Bit Operations/Compare To Constant  relop===  const=0  OutDataTypeStr=boolean
      settings: AttributesFormatString=Operator: %<relop>\nConst: %<const>
  Compare to Constant1 : simulink/Logic and Bit Operations/Compare To Constant  relop===  const=1  OutDataTypeStr=boolean
      settings: AttributesFormatString=Operator: %<relop>\nConst: %<const>
  Delay : Delay  DelayLength=1
  Logical Operator : Logic
  Out : Outport
  wires:
  Compare to Constant1/1 -> Logical Operator/1
  Delay/1 -> Compare to Constant/1
  Compare to Constant/1 -> Logical Operator/2
  Logical Operator/1 -> Out/1
  In/1 -> Delay/1, Compare to Constant1/1

== matlab function Tip-Off Assist Payload/Pseudo-Frictionless Weigh/MATLAB Function ==
  data: inputsBad input double; latched input double; status output double; measCondOk input double
function status = pfwStatus(inputsBad, latched, measCondOk)

if inputsBad
    status = TipAssistPfwStatus_t.FAULT;
elseif latched && measCondOk
    % Let consumers know that PFW is valid and may improve in confidence
    status = TipAssistPfwStatus_t.VALID_MEASURING;
elseif latched && ~measCondOk
    % Let consumers know that PFW is valid, but won't improve in confidence
    status = TipAssistPfwStatus_t.VALID_NOT_MEASURING;
elseif ~latched && measCondOk
    % Let consumers know that PFW is likely about to become valid
    status = TipAssistPfwStatus_t.PENDING;
else
    status = TipAssistPfwStatus_t.INVALID;
end

== matlab function Tip-Off Assist Payload/Weighing Statistics/Two Sided Confidence Limit ==
  data: confidence input double; bound output double; stdev input double
function bound = TwoSidedConfBound(confidence, stdev)
% Calculates the size of a confidence interval in terms of half its width.
%
% Inputs:
%   confidence
%   Confidence that the resulting bound will enclose the true value.
%
%   stdev
%   The observed standard deviation, expressed in the same units as
%   bound. Can be thought of as defining the scale of the normal
%   distribution that we are assuming represents the data we are sampling.
%
%   Potential units for the arguments are percent of rated payload or
%   payload.
%
% Outputs:
%   bound
%   Bound of the confidence interval, expressed in the same units as stdev.
%   
%   For lower bound, the true value will lie above the mean minus this
%   value.
%   The opposite is true for an upper bound.
%   
% Inspired from pcs_calculate_confidence() in pcs_io.c

% Table of confidence vs two-sided confidence interval bound.
% Units of confidence decimal percent and the ratio of standard
% deviation of a standard normal distribution.
xConfidenceTwoSided = [ 0.0, 0.235822844, 0.382924922, 0.516072694, 0.631879747, 0.728667676, 0.806398927, 0.866385543, 0.910869057, 0.942566872, 0.964271153, 0.978551778, 0.987580668, 0.993066052, 0.997300204, 0.999534742, 1.0 ];
yStdevRatio = [ 0.0, 0.3, 0.5, 0.7, 0.9, 1.1, 1.3, 1.5, 1.7, 1.9, 2.1, 2.3, 2.5, 2.7, 3.0, 3.5, 4.0 ];
stdev_ratio = interp1(xConfidenceTwoSided, yStdevRatio, confidence);
bound = stdev_ratio * stdev;

== matlab function Tip-Off Assist Payload/Weighing Statistics/One Sided Confidence Limit ==
  data: confidence input double; bound output double; stdev input double
function bound = oneSidedConfBound(confidence, stdev)
% Calculates the size of a confidence interval in terms of half its width.
%
% Inputs:
%   confidence
%   Confidence that the resulting bound will enclose the true value.
%
%   stdev
%   The observed standard deviation, expressed in the same units as
%   bound. Can be thought of as defining the scale of the normal
%   distribution that we are assuming represents the data we are sampling.
%
%   Potential units for the arguments are percent of rated payload or
%   payload.
%
% Outputs:
%   bound
%   Bound of the confidence interval, expressed in the same units as stdev.
%   
%   For lower bound, the true value will lie above the mean minus this
%   value.
%   The opposite is true for an upper bound.
%   
% Inspired from pcs_calculate_confidence() in pcs_io.c

% Table of confidence vs one-sided confidence interval bound.
% Units of confidence decimal percent and the ratio of standard
% deviation of a standard normal distribution.
xConfidenceOneSided = [0.500000000000000,0.617911422000000,0.691462461000000,0.758036347000000,0.815939873500000,0.864333838000000,0.903199463500000,0.933192771500000,0.955434528500000,0.971283436000000,0.982135576500000,0.989275889000000,0.993790334000000,0.996533026000000,0.998650102000000,0.999767371000000,1];
yStdevRatio = [ 0.0, 0.3, 0.5, 0.7, 0.9, 1.1, 1.3, 1.5, 1.7, 1.9, 2.1, 2.3, 2.5, 2.7, 3.0, 3.5, 4.0 ];
stdev_ratio = interp1(xConfidenceOneSided, yStdevRatio, confidence);
bound = stdev_ratio * stdev;

== matlab function EEF IMU to NEEF gravity vector/EEF vector to NEEF vector ==
  data: eefVector input double; neefVector output double; steeringAngle input double
function neefVector  = fcn(eefVector, steeringAngle)
% Transforms a vector on the EEF to a vector on the NEEF via steering angle
rotAxis = [0; 1; 0];               % Steering right is positive angle
angle = steeringAngle;

% Form rotation matrix
crossProductMatrix = [
    0,          -rotAxis(3),  rotAxis(2);
     rotAxis(3), 0,          -rotAxis(1);
    -rotAxis(2), rotAxis(1),  0
];
tensorProduct = rotAxis * transpose(rotAxis);
rotMatrix = cos(angle) * eye(3) + sin(angle) * crossProductMatrix + ...
    (1 - cos(angle)) * tensorProduct;

neefVector = rotMatrix * eefVector;

== matlab function EEF IMU to NEEF gravity vector/Rotation Matrix About Z ==
  data: angle input double; rotMatrix output double
function rotMatrix = fcn(angle)
% Calculates a rotation matrix from an angle in deg
if angle == 0
    rotMatrix = single(eye(3));
    return
end

angleRad = angle / 180.0 * pi;

% Form rotation matrix
a = cos(angleRad);
b = sin(angleRad);
rotMatrix = [
    a, -b, 0;
    b, a, 0;
    0, 0, 1
    ];

== matlab function EEF IMU to NEEF gravity vector/euler angles from rot matrix ==
  data: rotations output double; rotMatrix input double
function rotations  = decomp(rotMatrix)
%   Input:  3x3 rotation matrix
%   Output: 1x3 vector of euler angles in degrees
rotations = zeros(1,3);
rotations(1) = atan2(rotMatrix(3,2),rotMatrix(3,3));
rotations(2) = atan2(-rotMatrix(3,1), (sqrt((rotMatrix(3,2)^2)+(rotMatrix(3,3)^2))));
rotations(3) = atan2(rotMatrix(2,1),rotMatrix(1,1));
% convert back to degrees
for i=1:size(rotations,2)
    rotations(i) = 180*rotations(i)/pi;
end
end

== matlab function EEF IMU to NEEF gravity vector/rotation matrix calc from two vectors ==
  data: level_vec_meas input double; rotMatrix output double; level_vec_act input double; rotAxis output double; angle output double
function [rotMatrix, rotAxis, angle] = fcn(level_vec_meas, level_vec_act)
% Should match output of:
%     vrrotvec2mat(vrrotvec(level_vec_meas, level_vec_act))

if all(level_vec_meas == level_vec_act)
    % No transform necessary, return identity matrix
    rotAxis = single([9999; 9999; 9999]);
    angle = single(9999);
    rotMatrix = single(eye(3));
    return
end
    
a = level_vec_meas;
b = level_vec_act;

cp = cross(a, b);
cpNorm = norm(cp);

rotAxis = cp/cpNorm;
angle_rad = atan(cpNorm/dot(a, b));
angle = angle_rad * 180.0 / pi;

% Form rotation matrix
crossProductMatrix = [
    0,          -rotAxis(3),  rotAxis(2);
     rotAxis(3), 0,          -rotAxis(1);
    -rotAxis(2), rotAxis(1),  0
];
tensorProduct = rotAxis * transpose(rotAxis);
rotMatrix = cos(angle_rad) * eye(3) + sin(angle_rad) * crossProductMatrix + ...
    (1 - cos(angle_rad)) * tensorProduct;

== matlab function CPM Payload Send For when bucket is not racked/MATLAB Function ==
  data: pfwStatus input double; pfwPayload input double; outPayload output double; liveStatus input double; livePayload input double; outStatus output double
function [outPayload, outStatus]= sendCpmStatus(pfwStatus, pfwPayload, liveStatus, livePayload)

if pfwStatus == TipAssistPfwStatus_t.VALID_MEASURING || pfwStatus == TipAssistPfwStatus_t.VALID_NOT_MEASURING
	outStatus = TipAssistSendCpmStatus_t.PSEUDO_FRICTIONLESS;
    outPayload = pfwPayload;
elseif liveStatus == TipAssistLiveWeighStatus_t.VALID
    outStatus = TipAssistSendCpmStatus_t.LIVE;
    outPayload = livePayload;
else
    outStatus = TipAssistSendCpmStatus_t.INVALID;
    outPayload = single(NaN);
end

== matlab function Tip-Off Assist Payload/Pseudo-Frictionless Weigh/Weighing Statistics/One Sided Confidence Limit ==
  data: confidence input double; bound output double; stdev input double
function bound = oneSidedConfBound(confidence, stdev)
% Calculates the size of a confidence interval in terms of half its width.
%
% Inputs:
%   confidence
%   Confidence that the resulting bound will enclose the true value.
%
%   stdev
%   The observed standard deviation, expressed in the same units as
%   bound. Can be thought of as defining the scale of the normal
%   distribution that we are assuming represents the data we are sampling.
%
%   Potential units for the arguments are percent of rated payload or
%   payload.
%
% Outputs:
%   bound
%   Bound of the confidence interval, expressed in the same units as stdev.
%   
%   For lower bound, the true value will lie above the mean minus this
%   value.
%   The opposite is true for an upper bound.
%   
% Inspired from pcs_calculate_confidence() in pcs_io.c

% Table of confidence vs one-sided confidence interval bound.
% Units of confidence decimal percent and the ratio of standard
% deviation of a standard normal distribution.
xConfidenceOneSided = [0.500000000000000,0.617911422000000,0.691462461000000,0.758036347000000,0.815939873500000,0.864333838000000,0.903199463500000,0.933192771500000,0.955434528500000,0.971283436000000,0.982135576500000,0.989275889000000,0.993790334000000,0.996533026000000,0.998650102000000,0.999767371000000,1];
yStdevRatio = [ 0.0, 0.3, 0.5, 0.7, 0.9, 1.1, 1.3, 1.5, 1.7, 1.9, 2.1, 2.3, 2.5, 2.7, 3.0, 3.5, 4.0 ];
stdev_ratio = interp1(xConfidenceOneSided, yStdevRatio, confidence);
bound = stdev_ratio * stdev;

== matlab function Tip-Off Assist Payload/Pseudo-Frictionless Weigh/Weighing Statistics/Two Sided Confidence Limit ==
  data: confidence input double; bound output double; stdev input double
function bound = TwoSidedConfBound(confidence, stdev)
% Calculates the size of a confidence interval in terms of half its width.
%
% Inputs:
%   confidence
%   Confidence that the resulting bound will enclose the true value.
%
%   stdev
%   The observed standard deviation, expressed in the same units as
%   bound. Can be thought of as defining the scale of the normal
%   distribution that we are assuming represents the data we are sampling.
%
%   Potential units for the arguments are percent of rated payload or
%   payload.
%
% Outputs:
%   bound
%   Bound of the confidence interval, expressed in the same units as stdev.
%   
%   For lower bound, the true value will lie above the mean minus this
%   value.
%   The opposite is true for an upper bound.
%   
% Inspired from pcs_calculate_confidence() in pcs_io.c

% Table of confidence vs two-sided confidence interval bound.
% Units of confidence decimal percent and the ratio of standard
% deviation of a standard normal distribution.
xConfidenceTwoSided = [ 0.0, 0.235822844, 0.382924922, 0.516072694, 0.631879747, 0.728667676, 0.806398927, 0.866385543, 0.910869057, 0.942566872, 0.964271153, 0.978551778, 0.987580668, 0.993066052, 0.997300204, 0.999534742, 1.0 ];
yStdevRatio = [ 0.0, 0.3, 0.5, 0.7, 0.9, 1.1, 1.3, 1.5, 1.7, 1.9, 2.1, 2.3, 2.5, 2.7, 3.0, 3.5, 4.0 ];
stdev_ratio = interp1(xConfidenceTwoSided, yStdevRatio, confidence);
bound = stdev_ratio * stdev;
